simulink model "propulsion_system_test"  (R2026b)
settings: Solver=ode4  FixedStep=0.005
undefined symbols (not defined in the file): Ah, APC_alpha_deg, APC_Cd, APC_Cl, chord_distribution, eta_ESC, I_0, I_max, K_e, K_t, K_u, n_cells, n_motors, R_batt, R_m, radial_edges, rho_kgpm3, twist_distribution_deg
libraries: aerolibanimutils x1
settings Model: Creator=Teama  LastModifiedBy=Teama

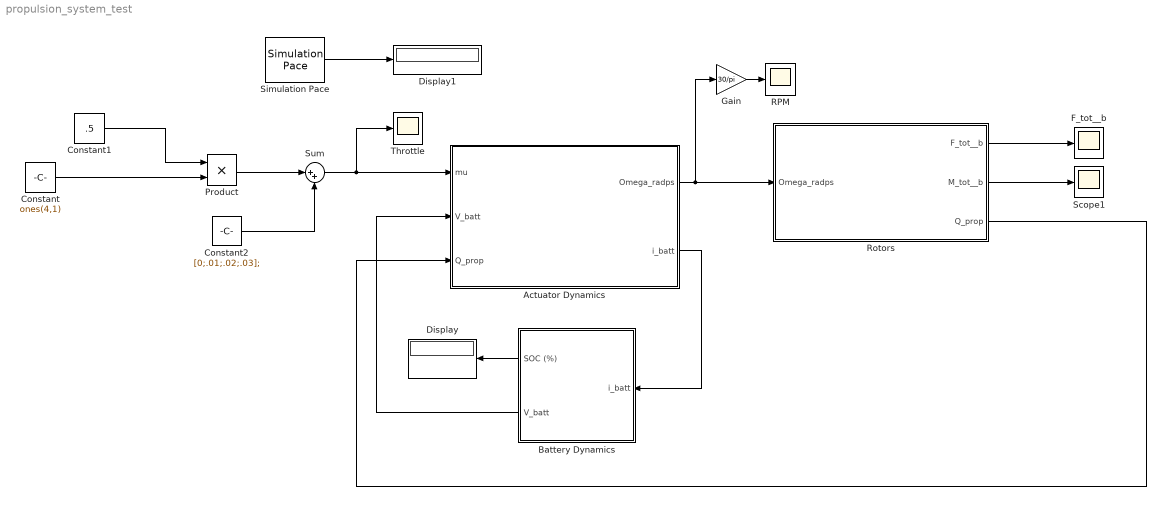
== system propulsion_system_test ==
  Actuator Dynamics : Subsystem
  Battery Dynamics : Subsystem
  Constant : Constant  Value=ones(4,1)
  Constant1 : Constant  Value=.5
  Constant2 : Constant  Value=[0;.01;.02;.03];
  Display : Display
  Display1 : Display
  F_tot__b : Scope
      settings: ActiveDisplayYMinimum=-8.2982783360854544  ActiveDisplayYMaximum=74.684505024769066
  Gain : Gain  Gain=30/pi
  Product : Product
  RPM : Scope
      settings: ActiveDisplayYMinimum=-185.85222226230545  ActiveDisplayYMaximum=3582.5293174634944  DataLoggingVariableName=ScopeData2
  Rotors : Subsystem
  Scope1 : Scope
  Simulation Pace : aerolibanimutils/Simulation Pace  SimulationPace=1  SleepMode=Auto  OutputPaceError=on  SampleTime=0.005
  Sum : Sum  Inputs=|++
  Throttle : Scope
      settings: ActiveDisplayYMinimum=0.49625  ActiveDisplayYMaximum=0.53375000000000006  DataLoggingVariableName=ScopeData3
  wires:
  Battery Dynamics/1(SOC (%)) -> Display/1
  Battery Dynamics/2(V_batt) -> Actuator Dynamics/2(V_batt)
  Constant/1 -> Product/2
  Rotors/1(F_tot__b) -> F_tot__b/1
  Rotors/2(M_tot__b) -> Scope1/1
  Rotors/3(Q_prop) -> Actuator Dynamics/3(Q_prop)
  Actuator Dynamics/2(i_batt) -> Battery Dynamics/1(i_batt)
  Actuator Dynamics/1(Omega_radps) -> Rotors/1(Omega_radps), Gain/1
  Simulation Pace/1 -> Display1/1
  Product/1 -> Sum/1
  Constant1/1 -> Product/1
  Sum/1 -> Throttle/1, Actuator Dynamics/1(mu)
  Constant2/1 -> Sum/2
  Gain/1 -> RPM/1

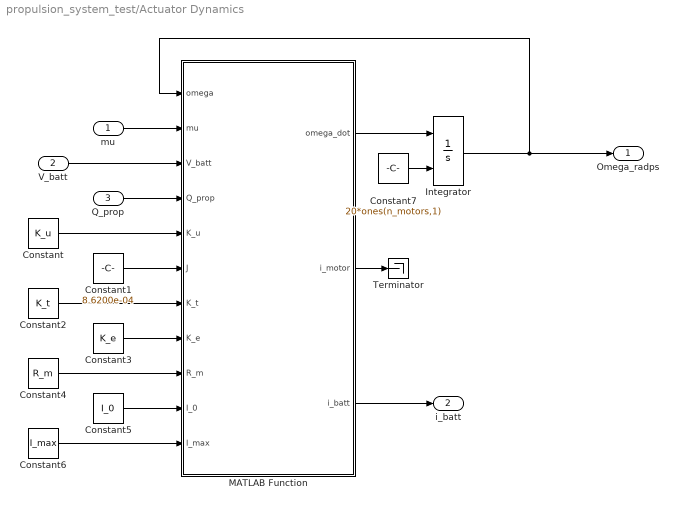
== system propulsion_system_test/Actuator Dynamics ==
  mu : Inport
  V_batt : Inport  Port=2
  Q_prop : Inport  Port=3
  Constant : Constant  Value=K_u
  Constant1 : Constant  Value=8.6200e-04
  Constant2 : Constant  Value=K_t
  Constant3 : Constant  Value=K_e
  Constant4 : Constant  Value=R_m
  Constant5 : Constant  Value=I_0
  Constant6 : Constant  Value=I_max
  Constant7 : Constant  Value=20*ones(n_motors,1)
  Integrator : Integrator  InitialConditionSource=external
  MATLAB Function : MATLAB Function  TreatAsAtomicUnit=on
  Terminator : Terminator
  Omega_radps : Outport
  i_batt : Outport  Port=2
  wires:
  mu/1 -> MATLAB Function/2(mu)
  MATLAB Function/1(omega_dot) -> Integrator/1
  Integrator/1 -> Omega_radps/1, MATLAB Function/1(omega)
  V_batt/1 -> MATLAB Function/3(V_batt)
  Q_prop/1 -> MATLAB Function/4(Q_prop)
  MATLAB Function/2(i_motor) -> Terminator/1
  MATLAB Function/3(i_batt) -> i_batt/1
  Constant/1 -> MATLAB Function/5(K_u)
  Constant1/1 -> MATLAB Function/6(J)
  Constant2/1 -> MATLAB Function/7(K_t)
  Constant3/1 -> MATLAB Function/8(K_e)
  Constant4/1 -> MATLAB Function/9(R_m)
  Constant5/1 -> MATLAB Function/10(I_0)
  Constant6/1 -> MATLAB Function/11(I_max)
  Constant7/1 -> Integrator/2

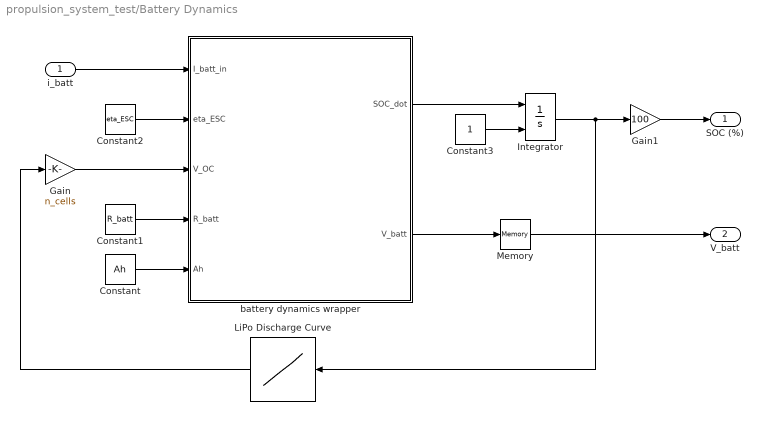
== system propulsion_system_test/Battery Dynamics ==
  i_batt : Inport
  Constant : Constant  Value=Ah
  Constant1 : Constant  Value=R_batt
  Constant2 : Constant  Value=eta_ESC
  Constant3 : Constant
  Gain : Gain  Gain=n_cells
  Gain1 : Gain  Gain=100
  Integrator : Integrator  InitialConditionSource=external
  LiPo Discharge Curve : Lookup_n-D  NumberOfTableDimensions=1  BreakpointsForDimension1="[0    0.05  0.10  0.20  0.30  0.40  0.50  0.60  0.70  0.80  0.90  1.00]"  Table="[3.20 3.45  3.55  3.65  3.70  3.74  3.77  3.80  3.84  3.90  4.00  4.20]"  InternalRulePriority=Speed  RndMeth=Simplest
  Memory : Memory  InitialCondition=4.2*n_cells
  battery dynamics wrapper : MATLAB Function  TreatAsAtomicUnit=on
  SOC (%) : Outport
  V_batt : Outport  Port=2
  wires:
  i_batt/1 -> battery dynamics wrapper/1(I_batt_in)
  battery dynamics wrapper/1(SOC_dot) -> Integrator/1
  Integrator/1 -> LiPo Discharge Curve/1, Gain1/1
  LiPo Discharge Curve/1 -> Gain/1
  Gain/1 -> battery dynamics wrapper/3(V_OC)
  battery dynamics wrapper/2(V_batt) -> Memory/1
  Gain1/1 -> SOC (%)/1
  Constant/1 -> battery dynamics wrapper/5(Ah)
  Constant1/1 -> battery dynamics wrapper/4(R_batt)
  Constant2/1 -> battery dynamics wrapper/2(eta_ESC)
  Memory/1 -> V_batt/1
  Constant3/1 -> Integrator/2

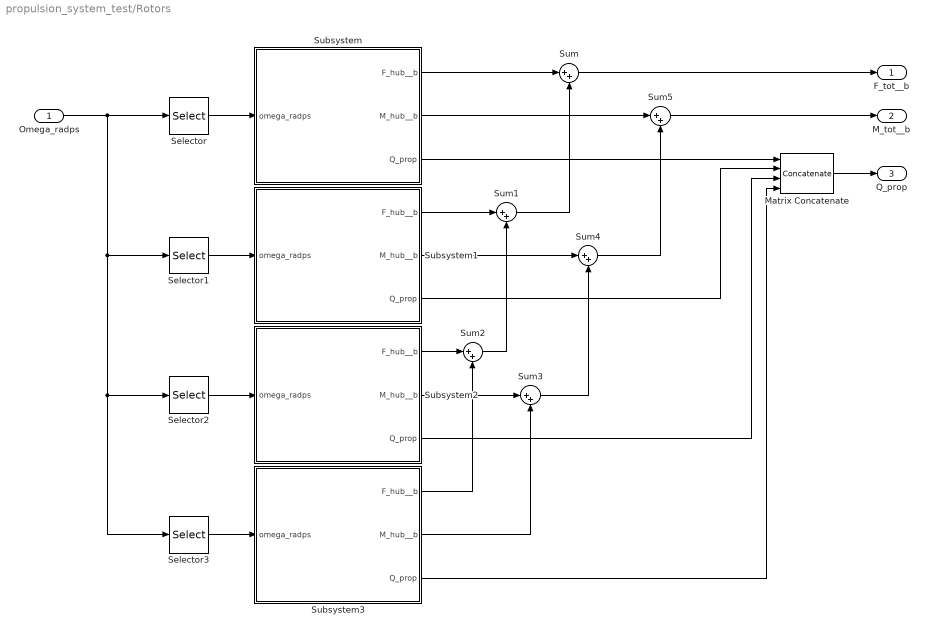
== system propulsion_system_test/Rotors ==
  Omega_radps : Inport
  Matrix Concatenate : Concatenate  NumInputs=4  Mode=Multidimensional array
  Selector : Selector  InputPortWidth=4  IndexOptions=Index vector (dialog)  Indices=[1]  OutputSizes=1
  Selector1 : Selector  InputPortWidth=4  IndexOptions=Index vector (dialog)  Indices=[2]  OutputSizes=1
  Selector2 : Selector  InputPortWidth=4  IndexOptions=Index vector (dialog)  Indices=[3]  OutputSizes=1
  Selector3 : Selector  InputPortWidth=4  IndexOptions=Index vector (dialog)  Indices=[4]  OutputSizes=1
  Subsystem : Subsystem
  Subsystem1 : Subsystem
  Subsystem2 : Subsystem
  Subsystem3 : Subsystem
  Sum{,1..5} (6 alike) : Sum  Inputs=|++
  F_tot__b : Outport
  M_tot__b : Outport  Port=2
  Q_prop : Outport  Port=3
  wires:
  Omega_radps/1 -> Selector3/1, Selector2/1, Selector1/1, Selector/1
  Subsystem/1(F_hub__b) -> Sum/1
  Subsystem/2(M_hub__b) -> Sum5/1
  Subsystem/3(Q_prop) -> Matrix Concatenate/1
  Selector/1 -> Subsystem/1(omega_radps)
  Selector1/1 -> Subsystem1/1(omega_radps)
  Selector2/1 -> Subsystem2/1(omega_radps)
  Selector3/1 -> Subsystem3/1(omega_radps)
  Subsystem3/1(F_hub__b) -> Sum2/2
  Subsystem2/1(F_hub__b) -> Sum2/1
  Sum1/1 -> Sum/2
  Subsystem1/1(F_hub__b) -> Sum1/1
  Sum2/1 -> Sum1/2
  Sum/1 -> F_tot__b/1
  Subsystem2/2(M_hub__b) -> Sum3/1
  Subsystem3/2(M_hub__b) -> Sum3/2
  Sum3/1 -> Sum4/2
  Subsystem1/2(M_hub__b) -> Sum4/1
  Sum4/1 -> Sum5/2
  Sum5/1 -> M_tot__b/1
  Subsystem1/3(Q_prop) -> Matrix Concatenate/2
  Subsystem2/3(Q_prop) -> Matrix Concatenate/3
  Subsystem3/3(Q_prop) -> Matrix Concatenate/4
  Matrix Concatenate/1 -> Q_prop/1

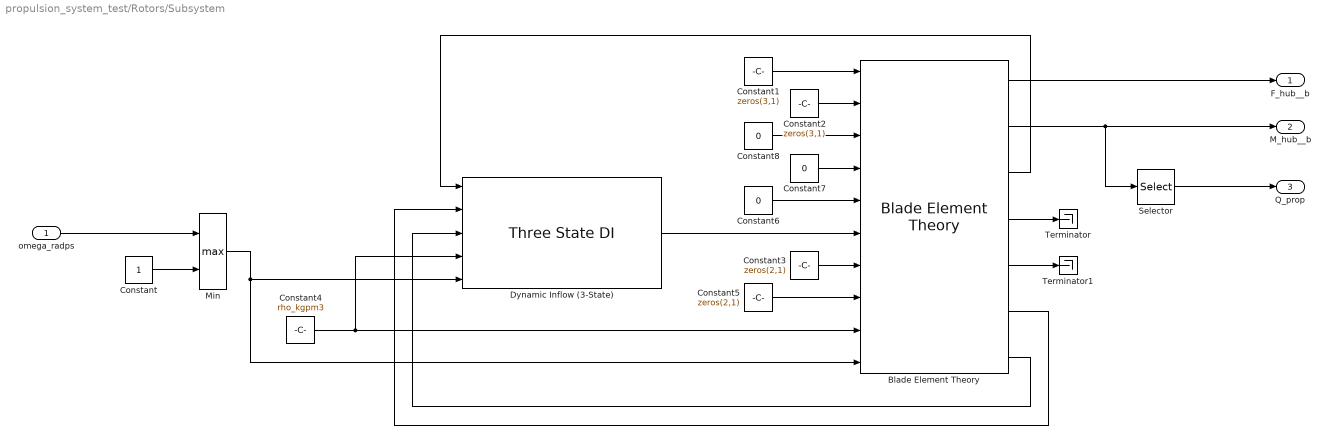
== system propulsion_system_test/Rotors/Subsystem ==
  omega_radps : Inport
  Blade Element Theory : BladeElementTheory  omegaSrc=Port  Nb=n_blades  radius=radius_m  bladeElements=radial_edges  outLoadDistribution=on  outVelocityRatio=on  chordDistribution=[radial_edges;chord_distribution]  twistType=Custom  twistDistribution=[radial_edges;twist_distribution_deg]  liftCoeffSpec=Lift coefficient matrix [α(deg); cl(non-dimensional)]  liftData=[APC_alpha_deg;APC_Cl]  dragCoeffSpec=Drag coefficient matrix [α(deg); cd(non-dimensional)]  dragData=[APC_alpha_deg;APC_Cd]
  Constant : Constant
  Constant1 : Constant  Value=zeros(3,1)
  Constant2 : Constant  Value=zeros(3,1)
  Constant3 : Constant  Value=zeros(2,1)
  Constant4 : Constant  Value=rho_kgpm3
  Constant5 : Constant  Value=zeros(2,1)
  Constant6 : Constant  Value=0
  Constant7 : Constant  Value=0
  Constant8 : Constant  Value=0
  Dynamic Inflow (3-State) : ThreeStateDI  omegaSrc=Port  radius=radius_m  radDistrSrc=Custom distribution  radDistr=radial_edges
  Min : MinMax  Function=max  Inputs=2
  Selector : Selector  InputPortWidth=3  IndexOptions=Index vector (dialog)  Indices=[3]  OutputSizes=1
  Terminator : Terminator
  Terminator1 : Terminator
  F_hub__b : Outport
  M_hub__b : Outport  Port=2
  Q_prop : Outport  Port=3
  wires:
  Constant8/1 -> Blade Element Theory/3
  Constant1/1 -> Blade Element Theory/1
  Constant2/1 -> Blade Element Theory/2
  Blade Element Theory/4 -> Terminator/1
  Constant7/1 -> Blade Element Theory/4
  Blade Element Theory/2 -> M_hub__b/1, Selector/1
  Constant6/1 -> Blade Element Theory/5
  Blade Element Theory/3 -> Dynamic Inflow (3-State)/1
  omega_radps/1 -> Min/1
  Dynamic Inflow (3-State)/1 -> Blade Element Theory/6
  Min/1 -> Blade Element Theory/10, Dynamic Inflow (3-State)/5
  Constant3/1 -> Blade Element Theory/7
  Blade Element Theory/5 -> Terminator1/1
  Constant/1 -> Min/2
  Constant5/1 -> Blade Element Theory/8
  Blade Element Theory/6 -> Dynamic Inflow (3-State)/2
  Constant4/1 -> Dynamic Inflow (3-State)/4, Blade Element Theory/9
  Blade Element Theory/7 -> Dynamic Inflow (3-State)/3
  Blade Element Theory/1 -> F_hub__b/1
  Selector/1 -> Q_prop/1

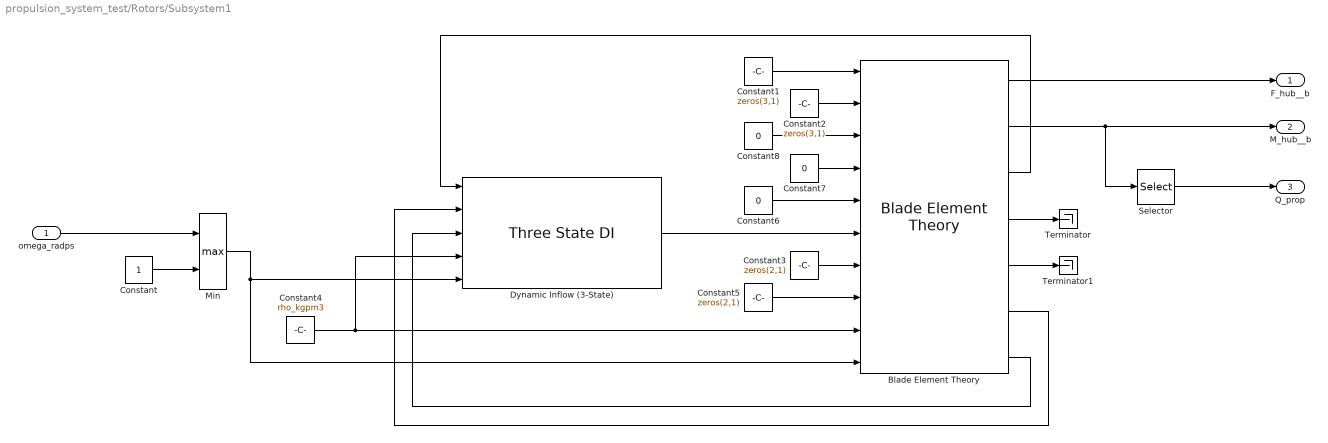
== system propulsion_system_test/Rotors/Subsystem1 ==
  omega_radps : Inport
  Blade Element Theory : BladeElementTheory  omegaSrc=Port  Nb=n_blades  radius=radius_m  bladeElements=radial_edges  outLoadDistribution=on  outVelocityRatio=on  chordDistribution=[radial_edges;chord_distribution]  twistType=Custom  twistDistribution=[radial_edges;twist_distribution_deg]  liftCoeffSpec=Lift coefficient matrix [α(deg); cl(non-dimensional)]  liftData=[APC_alpha_deg;APC_Cl]  dragCoeffSpec=Drag coefficient matrix [α(deg); cd(non-dimensional)]  dragData=[APC_alpha_deg;APC_Cd]
  Constant : Constant
  Constant1 : Constant  Value=zeros(3,1)
  Constant2 : Constant  Value=zeros(3,1)
  Constant3 : Constant  Value=zeros(2,1)
  Constant4 : Constant  Value=rho_kgpm3
  Constant5 : Constant  Value=zeros(2,1)
  Constant6 : Constant  Value=0
  Constant7 : Constant  Value=0
  Constant8 : Constant  Value=0
  Dynamic Inflow (3-State) : ThreeStateDI  omegaSrc=Port  radius=radius_m  radDistrSrc=Custom distribution  radDistr=radial_edges
  Min : MinMax  Function=max  Inputs=2
  Selector : Selector  InputPortWidth=3  IndexOptions=Index vector (dialog)  Indices=[3]  OutputSizes=1
  Terminator : Terminator
  Terminator1 : Terminator
  F_hub__b : Outport
  M_hub__b : Outport  Port=2
  Q_prop : Outport  Port=3
  wires:
  Selector/1 -> Q_prop/1
  Blade Element Theory/1 -> F_hub__b/1
  Blade Element Theory/7 -> Dynamic Inflow (3-State)/3
  Constant4/1 -> Blade Element Theory/9, Dynamic Inflow (3-State)/4
  Blade Element Theory/6 -> Dynamic Inflow (3-State)/2
  Constant5/1 -> Blade Element Theory/8
  Constant/1 -> Min/2
  Blade Element Theory/5 -> Terminator1/1
  Constant3/1 -> Blade Element Theory/7
  Min/1 -> Dynamic Inflow (3-State)/5, Blade Element Theory/10
  Dynamic Inflow (3-State)/1 -> Blade Element Theory/6
  omega_radps/1 -> Min/1
  Blade Element Theory/3 -> Dynamic Inflow (3-State)/1
  Constant6/1 -> Blade Element Theory/5
  Blade Element Theory/2 -> Selector/1, M_hub__b/1
  Constant7/1 -> Blade Element Theory/4
  Blade Element Theory/4 -> Terminator/1
  Constant2/1 -> Blade Element Theory/2
  Constant1/1 -> Blade Element Theory/1
  Constant8/1 -> Blade Element Theory/3

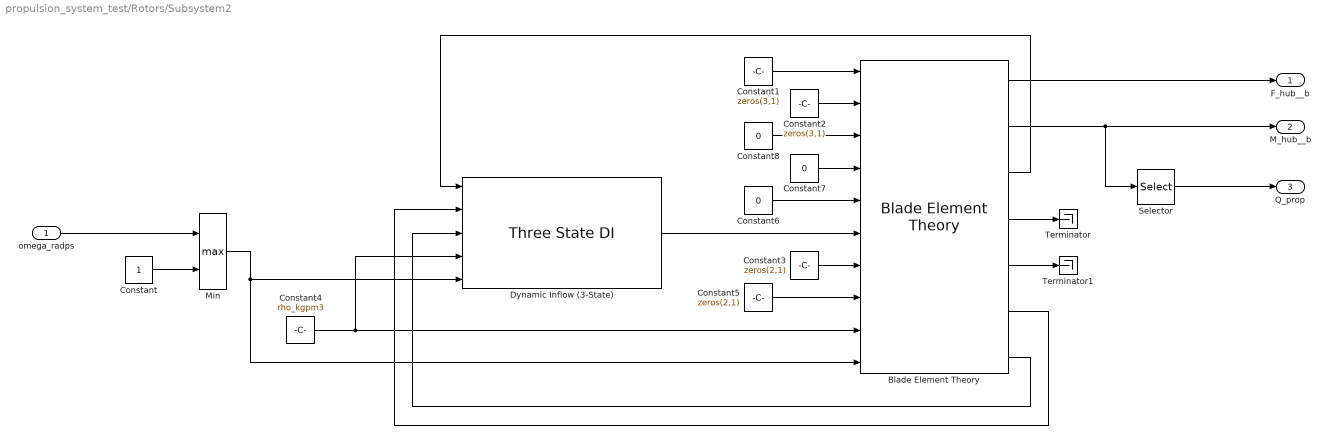
== system propulsion_system_test/Rotors/Subsystem2 ==
  omega_radps : Inport
  Blade Element Theory : BladeElementTheory  omegaSrc=Port  Nb=n_blades  radius=radius_m  bladeElements=radial_edges  outLoadDistribution=on  outVelocityRatio=on  chordDistribution=[radial_edges;chord_distribution]  twistType=Custom  twistDistribution=[radial_edges;twist_distribution_deg]  liftCoeffSpec=Lift coefficient matrix [α(deg); cl(non-dimensional)]  liftData=[APC_alpha_deg;APC_Cl]  dragCoeffSpec=Drag coefficient matrix [α(deg); cd(non-dimensional)]  dragData=[APC_alpha_deg;APC_Cd]
  Constant : Constant
  Constant1 : Constant  Value=zeros(3,1)
  Constant2 : Constant  Value=zeros(3,1)
  Constant3 : Constant  Value=zeros(2,1)
  Constant4 : Constant  Value=rho_kgpm3
  Constant5 : Constant  Value=zeros(2,1)
  Constant6 : Constant  Value=0
  Constant7 : Constant  Value=0
  Constant8 : Constant  Value=0
  Dynamic Inflow (3-State) : ThreeStateDI  omegaSrc=Port  radius=radius_m  radDistrSrc=Custom distribution  radDistr=radial_edges
  Min : MinMax  Function=max  Inputs=2
  Selector : Selector  InputPortWidth=3  IndexOptions=Index vector (dialog)  Indices=[3]  OutputSizes=1
  Terminator : Terminator
  Terminator1 : Terminator
  F_hub__b : Outport
  M_hub__b : Outport  Port=2
  Q_prop : Outport  Port=3
  wires:
  Constant8/1 -> Blade Element Theory/3
  Constant1/1 -> Blade Element Theory/1
  Constant2/1 -> Blade Element Theory/2
  Blade Element Theory/4 -> Terminator/1
  Constant7/1 -> Blade Element Theory/4
  Blade Element Theory/2 -> M_hub__b/1, Selector/1
  Constant6/1 -> Blade Element Theory/5
  Blade Element Theory/3 -> Dynamic Inflow (3-State)/1
  omega_radps/1 -> Min/1
  Dynamic Inflow (3-State)/1 -> Blade Element Theory/6
  Min/1 -> Blade Element Theory/10, Dynamic Inflow (3-State)/5
  Constant3/1 -> Blade Element Theory/7
  Blade Element Theory/5 -> Terminator1/1
  Constant/1 -> Min/2
  Constant5/1 -> Blade Element Theory/8
  Blade Element Theory/6 -> Dynamic Inflow (3-State)/2
  Constant4/1 -> Dynamic Inflow (3-State)/4, Blade Element Theory/9
  Blade Element Theory/7 -> Dynamic Inflow (3-State)/3
  Blade Element Theory/1 -> F_hub__b/1
  Selector/1 -> Q_prop/1

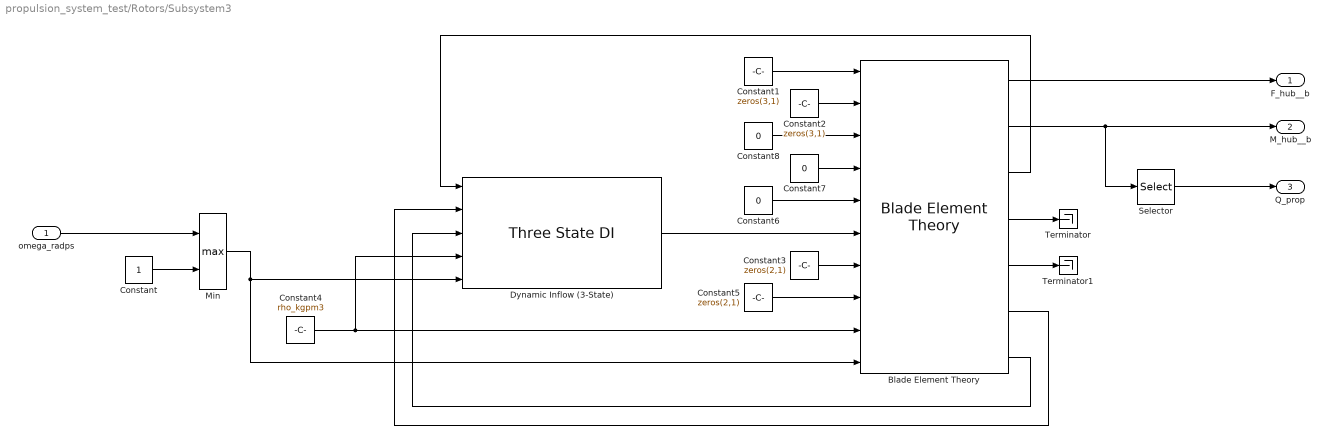
== system propulsion_system_test/Rotors/Subsystem3 ==
  omega_radps : Inport
  Blade Element Theory : BladeElementTheory  omegaSrc=Port  Nb=n_blades  radius=radius_m  bladeElements=radial_edges  outLoadDistribution=on  outVelocityRatio=on  chordDistribution=[radial_edges;chord_distribution]  twistType=Custom  twistDistribution=[radial_edges;twist_distribution_deg]  liftCoeffSpec=Lift coefficient matrix [α(deg); cl(non-dimensional)]  liftData=[APC_alpha_deg;APC_Cl]  dragCoeffSpec=Drag coefficient matrix [α(deg); cd(non-dimensional)]  dragData=[APC_alpha_deg;APC_Cd]
  Constant : Constant
  Constant1 : Constant  Value=zeros(3,1)
  Constant2 : Constant  Value=zeros(3,1)
  Constant3 : Constant  Value=zeros(2,1)
  Constant4 : Constant  Value=rho_kgpm3
  Constant5 : Constant  Value=zeros(2,1)
  Constant6 : Constant  Value=0
  Constant7 : Constant  Value=0
  Constant8 : Constant  Value=0
  Dynamic Inflow (3-State) : ThreeStateDI  omegaSrc=Port  radius=radius_m  radDistrSrc=Custom distribution  radDistr=radial_edges
  Min : MinMax  Function=max  Inputs=2
  Selector : Selector  InputPortWidth=3  IndexOptions=Index vector (dialog)  Indices=[3]  OutputSizes=1
  Terminator : Terminator
  Terminator1 : Terminator
  F_hub__b : Outport
  M_hub__b : Outport  Port=2
  Q_prop : Outport  Port=3
  wires:
  Selector/1 -> Q_prop/1
  Blade Element Theory/1 -> F_hub__b/1
  Blade Element Theory/7 -> Dynamic Inflow (3-State)/3
  Constant4/1 -> Blade Element Theory/9, Dynamic Inflow (3-State)/4
  Blade Element Theory/6 -> Dynamic Inflow (3-State)/2
  Constant5/1 -> Blade Element Theory/8
  Constant/1 -> Min/2
  Blade Element Theory/5 -> Terminator1/1
  Constant3/1 -> Blade Element Theory/7
  Min/1 -> Dynamic Inflow (3-State)/5, Blade Element Theory/10
  Dynamic Inflow (3-State)/1 -> Blade Element Theory/6
  omega_radps/1 -> Min/1
  Blade Element Theory/3 -> Dynamic Inflow (3-State)/1
  Constant6/1 -> Blade Element Theory/5
  Blade Element Theory/2 -> Selector/1, M_hub__b/1
  Constant7/1 -> Blade Element Theory/4
  Blade Element Theory/4 -> Terminator/1
  Constant2/1 -> Blade Element Theory/2
  Constant1/1 -> Blade Element Theory/1
  Constant8/1 -> Blade Element Theory/3

== matlab function propulsion_system_test/Battery Dynamics/battery dynamics wrapper ==
  data: I_batt_in input; eta_ESC input; SOC_dot output; V_OC input; R_batt input; Ah input; V_batt output
function [SOC_dot, V_batt] = battery_dynamics_wrapper(I_batt_in, eta_ESC, V_OC, R_batt, Ah)
    % initialize outputs
    I_batt_out = 0;
    SOC_dot = 0;

    [V_batt,~,~,SOC_dot] = battery_dynamics(I_batt_in, eta_ESC, V_OC, R_batt, Ah);
end

== matlab function propulsion_system_test/Actuator Dynamics/MATLAB Function ==
  data: omega input; mu input; omega_dot output size=[4,1]; V_batt input; Q_prop input; K_u input; J input; K_t input; K_e input; R_m input; I_0 input; I_max input; i_motor output double size=[4,1]; i_batt output double size=1
function [omega_dot, i_motor, i_batt] = motor_dynamics_wrapper(omega, mu, V_batt, Q_prop, K_u, J, K_t, K_e, R_m, I_0, I_max)
    [omega_dot, i_motor, i_batt] = motor_dynamics(mu, omega, V_batt, Q_prop, K_u, J, K_t, K_e, R_m, I_0, I_max);
end
